simulink model "Ten_phase_nine_leg_relocated_L3_L7"  (R2025b)
settings: Solver=VariableStepAuto  StartTime=0.0  StopTime=0.05  FixedStep=1e-6  MaxStep=1e-6  RelTol=1e-4
values from neighbouring files (symbols this model uses):
  bias_current = 5    [parameters_for_AMB_topology.m]
  half_SW_Ts = SW_Ts*0.5    (= 2.5e-05)    [parameters_for_AMB_topology.m]
  K_i = 2*pi*f_c*R_value/U_dc    (= 47.1238898038)    [parameters_for_AMB_topology.m]
  K_p = 2*pi*f_c*L_value/U_dc    (= 0.0235619449019)    [parameters_for_AMB_topology.m]
  R_value = 1    [parameters_for_AMB_topology.m]
  SW_Ts = 1/(SW_frequency)    (= 5e-05)    [parameters_for_AMB_topology.m]
libraries: fl_lib x61, simulink x39, nesl_utility x29, eeGeneralControl x28, ee_lib x19
(part 3 of 4)

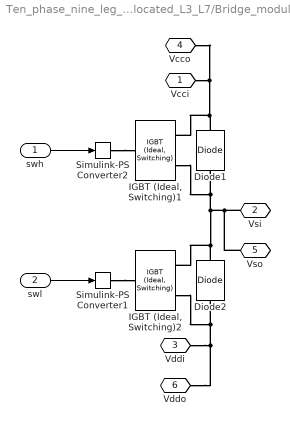
== system Ten_phase_nine_leg_relocated_L3_L7/Bridge_module6 ==
  swh : Inport
  swl : Inport  Port=2
  Diode1 : fl_lib/Electrical/Electrical Elements/Diode  Vf=0.6 V  Ron=0.3 Ohm  Goff=1e-8 1/Ohm  i_specify=off  i_priority=None  i=0 A  i_nominal_specify=off  i_nominal_value=1  i_nominal_unit=A  v_specify=off  v_priority=None  v=0 V  v_nominal_specify=off  v_nominal_value=1  v_nominal_unit=V
  Diode2 : fl_lib/Electrical/Electrical Elements/Diode  Vf=0.6 V  Ron=0.3 Ohm  Goff=1e-8 1/Ohm  i_specify=off  i_priority=None  i=0 A  i_nominal_specify=off  i_nominal_value=1  i_nominal_unit=A  v_specify=off  v_priority=None  v=0 V  v_nominal_specify=off  v_nominal_value=1  v_nominal_unit=V
  "IGBT (Ideal, Switching)1" : ee_lib/Semiconductors & Converters/IGBT (Ideal, Switching)  port_option=ee.enum.controlport.ps  Vf=0.8 V  Ron=0.001 Ohm  Goff=1e-5 1/Ohm  Vth=6 V  diode_param=ee.enum.semiconductors.protectionDiode.external  diode_Vf=0.8 V  diode_Ron=0.001 Ohm  diode_Goff=1e-5 1/Ohm  diode_C=50e-9 F  diode_iRM=-235 A  diode_iF=300 A  diode_idot=-50 A/us  diode_trr_param=ee.enum.converters.diodeReverseParam.trr_factor  diode_trr_factor=3  diode_trr=15 us  diode_Qrr=1500 s*uA  ice_specify=off  ice_priority=None  ice=0 A  ice_nominal_specify=off  ice_nominal_value=1  ice_nominal_unit=A  vce_specify=off  vce_priority=None  vce=0 V  vce_nominal_specify=off  vce_nominal_value=1  vce_nominal_unit=V  vge_specify=off  vge_priority=None  vge=0 V  vge_nominal_specify=off  vge_nominal_value=1  vge_nominal_unit=V  thermal_loss_option=ee.enum.converters.thermalLossOption.constantvalues  Von_data=[0, .1, .6, .8, 1, 1.3, 1.6, 2, 2.4; 0, .1, .7, 1, 1.2, 1.5, 1.9, 2.4, 2.8] V  Tj=[298.15, 398.15] K  Iout_data=[0, .1, 1, 5, 10, 20, 40, 70, 100] A  Eon_data=[0, .0024, .024, .12, .2, .48, 1.04, 2.16, 3.24; 0, .003, .03, .15, .25, .6, 1.3, 2.7, 4.05] * 1e-3 J  Eoff_data=[0, .0007, .0066, .033, .066, .17, .33, .83, 1.5; 0, .001, .01, .05, .1, .25, .5, 1.2, 2.2] * 1e-3 J  Eon_data_3D=[zeros(2, 9, 3)] J  Eoff_data_3D=[zeros(2, 9, 3)] J  Tj_loss=[298.15, 398.15] K  Iout_data_loss=[0, .1, 1, 5, 10, 20, 40, 70, 100] A  tabulateWithVce=false  Vce_loss=[0, 150, 300] V  Eon_scalar=22.86e-3 J  Eoff_scalar=17.14e-3 J  Voff=300 V  Iout_scalar=600 A  useCurrentFromPreviousCycle=false  useVoltageFromPreviousCycle=false  diodeModelType=ee.enum.converters.diodeModelType.pwl  diodeTableType=ee.enum.diode.tableType.IfMat  diode_ReverseIVType=ee.enum.diode.diodeReverseIV.constant  diode_IfMat=[.07, .12, .19, 1.75, 4.24, 7.32, 11.2; .16, .3, .72, 2.14, 4.02, 6.35, 9.12] A  diode_VfMat=[.9, 1.15, 1.25, 1.5, 1.75, 2.17, 2.6, 2.85; .58, .68, .75, 1.1, 1.38, 1.77, 2.27, 2.7] V  diode_TjVec=[25, 125] degC  diode_VfVec=[.5, .7, .9, 1.3, 1.7, 2.1, 2.5] V  diode_IfVec=[.1, .2, .5, 1, 2, 4, 7, 10] A  diode_IrMat=[1e-06, 2e-06, 5e-06, 1e-05, 2.5e-05, 5e-05, .0001; 2e-06, 5e-06, 1e-05, 4e-05, 8e-05, .0002, .0005] A  diode_VrMat=[10, 100, 200, 250, 300, 325, 350; 10, 70, 160, 220, 270, 300, 320] V  diode_VrVec=[10, 20, 40, 50, 70, 80, 100] V  diode_IrVec=[1e-06, 2e-06, 5e-06, 1e-05, 2e-05, 5e-05, .0001] A  diode_Vr=-600 V  diode_Ls=150 nH  diode_Erec=0.03 J  diode_rec_loss_model=ee.enum.diode.reverseRecoveryModel.fixed  diode_ErecVal=0 J  diode_scaleWithIandV=true  diode_ErecMat=zeros(2, 3) J  diode_TjrecVec=[298.15, 398.15] K  diode_IfrecVec=[.1, 1, 10] A  diode_IrecVal=10 A  diode_VrecVal=10 V  diode_tFilter=1 / 1000 / 100 s  separateThermalPortForDiode=false  thermal_network_parameterization=ee.enum.thermalNetworkTopology.external  Rth=[.08, .5] K/W  Rth_Cauer=[.08, .1, .5] K/W  Rth_Foster=[.08, .14, .22, .16] K/W  thermal_mass_parameterization=ee.enum.thermalNetwork.timeconstant  thermal_mass=[.01, .5] J/K  thermal_mass_Cauer=[.01, .1, .5] J/K  thermal_mass_Foster=[.001, .005, .05, .5] J/K  thermal_time_constant=[.001, .2] s  thermal_time_constant_Cauer=[.001, .1, .2] s  thermal_time_constant_Foster=[7e-05, .0007, .01, .08] s  thermal_mass_initial_temperatures=[25, 25] degC  thermal_mass_initial_temperatures_Cauer=[25, 25, 25] degC  junction_thermal_mass=0.01 J/K  Tvec_initial_Foster=[25, 25, 25, 25] degC  RthDiode=[.03, .2] K/W  RthCauerDiode=[.03, .1, .2] K/W  RthFosterDiode=[.03, .2] K/W  thermalMassDiode=[3, 25] J/K  thermalMassCauerDiode=[3, 10, 25] J/K  thermalMassFosterDiode=[33, 50] J/K  thermalTauDiode=[.1, 5] s  thermalTauCauerDiode=[.1, 1, 5] s  thermalTauFosterDiode=[1, 10] s  thermalMassInitTempDiode=[25, 25] degC  thermalMassInitTempCauerDiode=[25, 25, 25] degC  junctionthermalMassDiode=0.1 J/K  TVecInitialFosterDiode=[25, 25, 25, 25] degC  no_thermal_network=0  IGBT_junction_temperature_specify=off  IGBT_junction_temperature_priority=None  IGBT_junction_temperature=25 degC  IGBT_junction_temperature_nominal_specify=off  IGBT_junction_temperature_nominal_value=1  IGBT_junction_temperature_nominal_unit=degC  diode_junction_temperature_specify=off  diode_junction_temperature_priority=None  diode_junction_temperature=25 degC  diode_junction_temperature_nominal_specify=off  diode_junction_temperature_nominal_value=1  diode_junction_temperature_nominal_unit=degC  Qj_specify=off  Qj_priority=None  Qj=0 W  Qj_nominal_specify=off  Qj_nominal_value=1  Qj_nominal_unit=W  accumulatedSwitchingLosses_specify=off  accumulatedSwitchingLosses_priority=None  accumulatedSwitchingLosses=0 J
  "IGBT (Ideal, Switching)2" : ee_lib/Semiconductors & Converters/IGBT (Ideal, Switching)  port_option=ee.enum.controlport.ps  Vf=0.8 V  Ron=0.001 Ohm  Goff=1e-5 1/Ohm  Vth=6 V  diode_param=ee.enum.semiconductors.protectionDiode.external  diode_Vf=0.8 V  diode_Ron=0.001 Ohm  diode_Goff=1e-5 1/Ohm  diode_C=50e-9 F  diode_iRM=-235 A  diode_iF=300 A  diode_idot=-50 A/us  diode_trr_param=ee.enum.converters.diodeReverseParam.trr_factor  diode_trr_factor=3  diode_trr=15 us  diode_Qrr=1500 s*uA  ice_specify=off  ice_priority=None  ice=0 A  ice_nominal_specify=off  ice_nominal_value=1  ice_nominal_unit=A  vce_specify=off  vce_priority=None  vce=0 V  vce_nominal_specify=off  vce_nominal_value=1  vce_nominal_unit=V  vge_specify=off  vge_priority=None  vge=0 V  vge_nominal_specify=off  vge_nominal_value=1  vge_nominal_unit=V  thermal_loss_option=ee.enum.converters.thermalLossOption.constantvalues  Von_data=[0, .1, .6, .8, 1, 1.3, 1.6, 2, 2.4; 0, .1, .7, 1, 1.2, 1.5, 1.9, 2.4, 2.8] V  Tj=[298.15, 398.15] K  Iout_data=[0, .1, 1, 5, 10, 20, 40, 70, 100] A  Eon_data=[0, .0024, .024, .12, .2, .48, 1.04, 2.16, 3.24; 0, .003, .03, .15, .25, .6, 1.3, 2.7, 4.05] * 1e-3 J  Eoff_data=[0, .0007, .0066, .033, .066, .17, .33, .83, 1.5; 0, .001, .01, .05, .1, .25, .5, 1.2, 2.2] * 1e-3 J  Eon_data_3D=[zeros(2, 9, 3)] J  Eoff_data_3D=[zeros(2, 9, 3)] J  Tj_loss=[298.15, 398.15] K  Iout_data_loss=[0, .1, 1, 5, 10, 20, 40, 70, 100] A  tabulateWithVce=false  Vce_loss=[0, 150, 300] V  Eon_scalar=22.86e-3 J  Eoff_scalar=17.14e-3 J  Voff=300 V  Iout_scalar=600 A  useCurrentFromPreviousCycle=false  useVoltageFromPreviousCycle=false  diodeModelType=ee.enum.converters.diodeModelType.pwl  diodeTableType=ee.enum.diode.tableType.IfMat  diode_ReverseIVType=ee.enum.diode.diodeReverseIV.constant  diode_IfMat=[.07, .12, .19, 1.75, 4.24, 7.32, 11.2; .16, .3, .72, 2.14, 4.02, 6.35, 9.12] A  diode_VfMat=[.9, 1.15, 1.25, 1.5, 1.75, 2.17, 2.6, 2.85; .58, .68, .75, 1.1, 1.38, 1.77, 2.27, 2.7] V  diode_TjVec=[25, 125] degC  diode_VfVec=[.5, .7, .9, 1.3, 1.7, 2.1, 2.5] V  diode_IfVec=[.1, .2, .5, 1, 2, 4, 7, 10] A  diode_IrMat=[1e-06, 2e-06, 5e-06, 1e-05, 2.5e-05, 5e-05, .0001; 2e-06, 5e-06, 1e-05, 4e-05, 8e-05, .0002, .0005] A  diode_VrMat=[10, 100, 200, 250, 300, 325, 350; 10, 70, 160, 220, 270, 300, 320] V  diode_VrVec=[10, 20, 40, 50, 70, 80, 100] V  diode_IrVec=[1e-06, 2e-06, 5e-06, 1e-05, 2e-05, 5e-05, .0001] A  diode_Vr=-600 V  diode_Ls=150 nH  diode_Erec=0.03 J  diode_rec_loss_model=ee.enum.diode.reverseRecoveryModel.fixed  diode_ErecVal=0 J  diode_scaleWithIandV=true  diode_ErecMat=zeros(2, 3) J  diode_TjrecVec=[298.15, 398.15] K  diode_IfrecVec=[.1, 1, 10] A  diode_IrecVal=10 A  diode_VrecVal=10 V  diode_tFilter=1 / 1000 / 100 s  separateThermalPortForDiode=false  thermal_network_parameterization=ee.enum.thermalNetworkTopology.external  Rth=[.08, .5] K/W  Rth_Cauer=[.08, .1, .5] K/W  Rth_Foster=[.08, .14, .22, .16] K/W  thermal_mass_parameterization=ee.enum.thermalNetwork.timeconstant  thermal_mass=[.01, .5] J/K  thermal_mass_Cauer=[.01, .1, .5] J/K  thermal_mass_Foster=[.001, .005, .05, .5] J/K  thermal_time_constant=[.001, .2] s  thermal_time_constant_Cauer=[.001, .1, .2] s  thermal_time_constant_Foster=[7e-05, .0007, .01, .08] s  thermal_mass_initial_temperatures=[25, 25] degC  thermal_mass_initial_temperatures_Cauer=[25, 25, 25] degC  junction_thermal_mass=0.01 J/K  Tvec_initial_Foster=[25, 25, 25, 25] degC  RthDiode=[.03, .2] K/W  RthCauerDiode=[.03, .1, .2] K/W  RthFosterDiode=[.03, .2] K/W  thermalMassDiode=[3, 25] J/K  thermalMassCauerDiode=[3, 10, 25] J/K  thermalMassFosterDiode=[33, 50] J/K  thermalTauDiode=[.1, 5] s  thermalTauCauerDiode=[.1, 1, 5] s  thermalTauFosterDiode=[1, 10] s  thermalMassInitTempDiode=[25, 25] degC  thermalMassInitTempCauerDiode=[25, 25, 25] degC  junctionthermalMassDiode=0.1 J/K  TVecInitialFosterDiode=[25, 25, 25, 25] degC  no_thermal_network=0  IGBT_junction_temperature_specify=off  IGBT_junction_temperature_priority=None  IGBT_junction_temperature=25 degC  IGBT_junction_temperature_nominal_specify=off  IGBT_junction_temperature_nominal_value=1  IGBT_junction_temperature_nominal_unit=degC  diode_junction_temperature_specify=off  diode_junction_temperature_priority=None  diode_junction_temperature=25 degC  diode_junction_temperature_nominal_specify=off  diode_junction_temperature_nominal_value=1  diode_junction_temperature_nominal_unit=degC  Qj_specify=off  Qj_priority=None  Qj=0 W  Qj_nominal_specify=off  Qj_nominal_value=1  Qj_nominal_unit=W  accumulatedSwitchingLosses_specify=off  accumulatedSwitchingLosses_priority=None  accumulatedSwitchingLosses=0 J
  Simulink-PS Converter1 : nesl_utility/Simulink-PS Converter  PhysicalDomain=network_engine_domain  SubClassName=ps_input  LeftPortType=input  RightPortType=output  PseudoPeriodic=off  Frequencies=[]  NoiseDistribution=none  NoiseParameters=[]  Unit=1  AffineConversion=off  FilteringAndDerivatives=provide  SimscapeFilterOrder=1  InputFilterTimeConstant=0.001  UdotUserProvided=0
  Simulink-PS Converter2 : nesl_utility/Simulink-PS Converter  PhysicalDomain=network_engine_domain  SubClassName=ps_input  LeftPortType=input  RightPortType=output  PseudoPeriodic=off  Frequencies=[]  NoiseDistribution=none  NoiseParameters=[]  Unit=1  AffineConversion=off  FilteringAndDerivatives=provide  SimscapeFilterOrder=1  InputFilterTimeConstant=0.001  UdotUserProvided=0
  Vcci : PMIOPort  Side=Left
  Vsi : PMIOPort  Port=2  Side=Left
  Vddi : PMIOPort  Port=3  Side=Left
  Vcco : PMIOPort  Port=4  Side=Right
  Vso : PMIOPort  Port=5  Side=Right
  Vddo : PMIOPort  Port=6  Side=Right
  wires:
  swh/1 -> Simulink-PS Converter2/1
  swl/1 -> Simulink-PS Converter1/1
  connections:
  Diode1/RConn1 -- Vcco/RConn1 -- Vcci/RConn1 -- "IGBT (Ideal, Switching)1"/RConn1
  Simulink-PS Converter2/RConn1 -- "IGBT (Ideal, Switching)1"/LConn1
  "IGBT (Ideal, Switching)1"/RConn2 -- Vso/RConn1 -- Vsi/RConn1 -- "IGBT (Ideal, Switching)2"/RConn1 -- Diode2/RConn1 -- Diode1/LConn1
  "IGBT (Ideal, Switching)2"/RConn2 -- Vddo/RConn1 -- Vddi/RConn1 -- Diode2/LConn1
  Simulink-PS Converter1/RConn1 -- "IGBT (Ideal, Switching)2"/LConn1

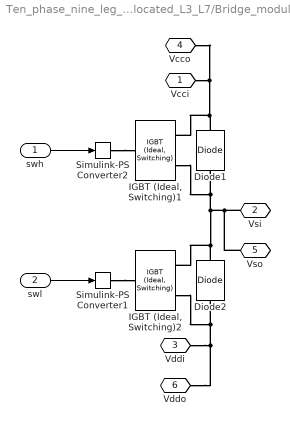
== system Ten_phase_nine_leg_relocated_L3_L7/Bridge_module7 ==
  swh : Inport
  swl : Inport  Port=2
  Diode1 : fl_lib/Electrical/Electrical Elements/Diode  Vf=0.6 V  Ron=0.3 Ohm  Goff=1e-8 1/Ohm  i_specify=off  i_priority=None  i=0 A  i_nominal_specify=off  i_nominal_value=1  i_nominal_unit=A  v_specify=off  v_priority=None  v=0 V  v_nominal_specify=off  v_nominal_value=1  v_nominal_unit=V
  Diode2 : fl_lib/Electrical/Electrical Elements/Diode  Vf=0.6 V  Ron=0.3 Ohm  Goff=1e-8 1/Ohm  i_specify=off  i_priority=None  i=0 A  i_nominal_specify=off  i_nominal_value=1  i_nominal_unit=A  v_specify=off  v_priority=None  v=0 V  v_nominal_specify=off  v_nominal_value=1  v_nominal_unit=V
  "IGBT (Ideal, Switching)1" : ee_lib/Semiconductors & Converters/IGBT (Ideal, Switching)  port_option=ee.enum.controlport.ps  Vf=0.8 V  Ron=0.001 Ohm  Goff=1e-5 1/Ohm  Vth=6 V  diode_param=ee.enum.semiconductors.protectionDiode.external  diode_Vf=0.8 V  diode_Ron=0.001 Ohm  diode_Goff=1e-5 1/Ohm  diode_C=50e-9 F  diode_iRM=-235 A  diode_iF=300 A  diode_idot=-50 A/us  diode_trr_param=ee.enum.converters.diodeReverseParam.trr_factor  diode_trr_factor=3  diode_trr=15 us  diode_Qrr=1500 s*uA  ice_specify=off  ice_priority=None  ice=0 A  ice_nominal_specify=off  ice_nominal_value=1  ice_nominal_unit=A  vce_specify=off  vce_priority=None  vce=0 V  vce_nominal_specify=off  vce_nominal_value=1  vce_nominal_unit=V  vge_specify=off  vge_priority=None  vge=0 V  vge_nominal_specify=off  vge_nominal_value=1  vge_nominal_unit=V  thermal_loss_option=ee.enum.converters.thermalLossOption.constantvalues  Von_data=[0, .1, .6, .8, 1, 1.3, 1.6, 2, 2.4; 0, .1, .7, 1, 1.2, 1.5, 1.9, 2.4, 2.8] V  Tj=[298.15, 398.15] K  Iout_data=[0, .1, 1, 5, 10, 20, 40, 70, 100] A  Eon_data=[0, .0024, .024, .12, .2, .48, 1.04, 2.16, 3.24; 0, .003, .03, .15, .25, .6, 1.3, 2.7, 4.05] * 1e-3 J  Eoff_data=[0, .0007, .0066, .033, .066, .17, .33, .83, 1.5; 0, .001, .01, .05, .1, .25, .5, 1.2, 2.2] * 1e-3 J  Eon_data_3D=[zeros(2, 9, 3)] J  Eoff_data_3D=[zeros(2, 9, 3)] J  Tj_loss=[298.15, 398.15] K  Iout_data_loss=[0, .1, 1, 5, 10, 20, 40, 70, 100] A  tabulateWithVce=false  Vce_loss=[0, 150, 300] V  Eon_scalar=22.86e-3 J  Eoff_scalar=17.14e-3 J  Voff=300 V  Iout_scalar=600 A  useCurrentFromPreviousCycle=false  useVoltageFromPreviousCycle=false  diodeModelType=ee.enum.converters.diodeModelType.pwl  diodeTableType=ee.enum.diode.tableType.IfMat  diode_ReverseIVType=ee.enum.diode.diodeReverseIV.constant  diode_IfMat=[.07, .12, .19, 1.75, 4.24, 7.32, 11.2; .16, .3, .72, 2.14, 4.02, 6.35, 9.12] A  diode_VfMat=[.9, 1.15, 1.25, 1.5, 1.75, 2.17, 2.6, 2.85; .58, .68, .75, 1.1, 1.38, 1.77, 2.27, 2.7] V  diode_TjVec=[25, 125] degC  diode_VfVec=[.5, .7, .9, 1.3, 1.7, 2.1, 2.5] V  diode_IfVec=[.1, .2, .5, 1, 2, 4, 7, 10] A  diode_IrMat=[1e-06, 2e-06, 5e-06, 1e-05, 2.5e-05, 5e-05, .0001; 2e-06, 5e-06, 1e-05, 4e-05, 8e-05, .0002, .0005] A  diode_VrMat=[10, 100, 200, 250, 300, 325, 350; 10, 70, 160, 220, 270, 300, 320] V  diode_VrVec=[10, 20, 40, 50, 70, 80, 100] V  diode_IrVec=[1e-06, 2e-06, 5e-06, 1e-05, 2e-05, 5e-05, .0001] A  diode_Vr=-600 V  diode_Ls=150 nH  diode_Erec=0.03 J  diode_rec_loss_model=ee.enum.diode.reverseRecoveryModel.fixed  diode_ErecVal=0 J  diode_scaleWithIandV=true  diode_ErecMat=zeros(2, 3) J  diode_TjrecVec=[298.15, 398.15] K  diode_IfrecVec=[.1, 1, 10] A  diode_IrecVal=10 A  diode_VrecVal=10 V  diode_tFilter=1 / 1000 / 100 s  separateThermalPortForDiode=false  thermal_network_parameterization=ee.enum.thermalNetworkTopology.external  Rth=[.08, .5] K/W  Rth_Cauer=[.08, .1, .5] K/W  Rth_Foster=[.08, .14, .22, .16] K/W  thermal_mass_parameterization=ee.enum.thermalNetwork.timeconstant  thermal_mass=[.01, .5] J/K  thermal_mass_Cauer=[.01, .1, .5] J/K  thermal_mass_Foster=[.001, .005, .05, .5] J/K  thermal_time_constant=[.001, .2] s  thermal_time_constant_Cauer=[.001, .1, .2] s  thermal_time_constant_Foster=[7e-05, .0007, .01, .08] s  thermal_mass_initial_temperatures=[25, 25] degC  thermal_mass_initial_temperatures_Cauer=[25, 25, 25] degC  junction_thermal_mass=0.01 J/K  Tvec_initial_Foster=[25, 25, 25, 25] degC  RthDiode=[.03, .2] K/W  RthCauerDiode=[.03, .1, .2] K/W  RthFosterDiode=[.03, .2] K/W  thermalMassDiode=[3, 25] J/K  thermalMassCauerDiode=[3, 10, 25] J/K  thermalMassFosterDiode=[33, 50] J/K  thermalTauDiode=[.1, 5] s  thermalTauCauerDiode=[.1, 1, 5] s  thermalTauFosterDiode=[1, 10] s  thermalMassInitTempDiode=[25, 25] degC  thermalMassInitTempCauerDiode=[25, 25, 25] degC  junctionthermalMassDiode=0.1 J/K  TVecInitialFosterDiode=[25, 25, 25, 25] degC  no_thermal_network=0  IGBT_junction_temperature_specify=off  IGBT_junction_temperature_priority=None  IGBT_junction_temperature=25 degC  IGBT_junction_temperature_nominal_specify=off  IGBT_junction_temperature_nominal_value=1  IGBT_junction_temperature_nominal_unit=degC  diode_junction_temperature_specify=off  diode_junction_temperature_priority=None  diode_junction_temperature=25 degC  diode_junction_temperature_nominal_specify=off  diode_junction_temperature_nominal_value=1  diode_junction_temperature_nominal_unit=degC  Qj_specify=off  Qj_priority=None  Qj=0 W  Qj_nominal_specify=off  Qj_nominal_value=1  Qj_nominal_unit=W  accumulatedSwitchingLosses_specify=off  accumulatedSwitchingLosses_priority=None  accumulatedSwitchingLosses=0 J
  "IGBT (Ideal, Switching)2" : ee_lib/Semiconductors & Converters/IGBT (Ideal, Switching)  port_option=ee.enum.controlport.ps  Vf=0.8 V  Ron=0.001 Ohm  Goff=1e-5 1/Ohm  Vth=6 V  diode_param=ee.enum.semiconductors.protectionDiode.external  diode_Vf=0.8 V  diode_Ron=0.001 Ohm  diode_Goff=1e-5 1/Ohm  diode_C=50e-9 F  diode_iRM=-235 A  diode_iF=300 A  diode_idot=-50 A/us  diode_trr_param=ee.enum.converters.diodeReverseParam.trr_factor  diode_trr_factor=3  diode_trr=15 us  diode_Qrr=1500 s*uA  ice_specify=off  ice_priority=None  ice=0 A  ice_nominal_specify=off  ice_nominal_value=1  ice_nominal_unit=A  vce_specify=off  vce_priority=None  vce=0 V  vce_nominal_specify=off  vce_nominal_value=1  vce_nominal_unit=V  vge_specify=off  vge_priority=None  vge=0 V  vge_nominal_specify=off  vge_nominal_value=1  vge_nominal_unit=V  thermal_loss_option=ee.enum.converters.thermalLossOption.constantvalues  Von_data=[0, .1, .6, .8, 1, 1.3, 1.6, 2, 2.4; 0, .1, .7, 1, 1.2, 1.5, 1.9, 2.4, 2.8] V  Tj=[298.15, 398.15] K  Iout_data=[0, .1, 1, 5, 10, 20, 40, 70, 100] A  Eon_data=[0, .0024, .024, .12, .2, .48, 1.04, 2.16, 3.24; 0, .003, .03, .15, .25, .6, 1.3, 2.7, 4.05] * 1e-3 J  Eoff_data=[0, .0007, .0066, .033, .066, .17, .33, .83, 1.5; 0, .001, .01, .05, .1, .25, .5, 1.2, 2.2] * 1e-3 J  Eon_data_3D=[zeros(2, 9, 3)] J  Eoff_data_3D=[zeros(2, 9, 3)] J  Tj_loss=[298.15, 398.15] K  Iout_data_loss=[0, .1, 1, 5, 10, 20, 40, 70, 100] A  tabulateWithVce=false  Vce_loss=[0, 150, 300] V  Eon_scalar=22.86e-3 J  Eoff_scalar=17.14e-3 J  Voff=300 V  Iout_scalar=600 A  useCurrentFromPreviousCycle=false  useVoltageFromPreviousCycle=false  diodeModelType=ee.enum.converters.diodeModelType.pwl  diodeTableType=ee.enum.diode.tableType.IfMat  diode_ReverseIVType=ee.enum.diode.diodeReverseIV.constant  diode_IfMat=[.07, .12, .19, 1.75, 4.24, 7.32, 11.2; .16, .3, .72, 2.14, 4.02, 6.35, 9.12] A  diode_VfMat=[.9, 1.15, 1.25, 1.5, 1.75, 2.17, 2.6, 2.85; .58, .68, .75, 1.1, 1.38, 1.77, 2.27, 2.7] V  diode_TjVec=[25, 125] degC  diode_VfVec=[.5, .7, .9, 1.3, 1.7, 2.1, 2.5] V  diode_IfVec=[.1, .2, .5, 1, 2, 4, 7, 10] A  diode_IrMat=[1e-06, 2e-06, 5e-06, 1e-05, 2.5e-05, 5e-05, .0001; 2e-06, 5e-06, 1e-05, 4e-05, 8e-05, .0002, .0005] A  diode_VrMat=[10, 100, 200, 250, 300, 325, 350; 10, 70, 160, 220, 270, 300, 320] V  diode_VrVec=[10, 20, 40, 50, 70, 80, 100] V  diode_IrVec=[1e-06, 2e-06, 5e-06, 1e-05, 2e-05, 5e-05, .0001] A  diode_Vr=-600 V  diode_Ls=150 nH  diode_Erec=0.03 J  diode_rec_loss_model=ee.enum.diode.reverseRecoveryModel.fixed  diode_ErecVal=0 J  diode_scaleWithIandV=true  diode_ErecMat=zeros(2, 3) J  diode_TjrecVec=[298.15, 398.15] K  diode_IfrecVec=[.1, 1, 10] A  diode_IrecVal=10 A  diode_VrecVal=10 V  diode_tFilter=1 / 1000 / 100 s  separateThermalPortForDiode=false  thermal_network_parameterization=ee.enum.thermalNetworkTopology.external  Rth=[.08, .5] K/W  Rth_Cauer=[.08, .1, .5] K/W  Rth_Foster=[.08, .14, .22, .16] K/W  thermal_mass_parameterization=ee.enum.thermalNetwork.timeconstant  thermal_mass=[.01, .5] J/K  thermal_mass_Cauer=[.01, .1, .5] J/K  thermal_mass_Foster=[.001, .005, .05, .5] J/K  thermal_time_constant=[.001, .2] s  thermal_time_constant_Cauer=[.001, .1, .2] s  thermal_time_constant_Foster=[7e-05, .0007, .01, .08] s  thermal_mass_initial_temperatures=[25, 25] degC  thermal_mass_initial_temperatures_Cauer=[25, 25, 25] degC  junction_thermal_mass=0.01 J/K  Tvec_initial_Foster=[25, 25, 25, 25] degC  RthDiode=[.03, .2] K/W  RthCauerDiode=[.03, .1, .2] K/W  RthFosterDiode=[.03, .2] K/W  thermalMassDiode=[3, 25] J/K  thermalMassCauerDiode=[3, 10, 25] J/K  thermalMassFosterDiode=[33, 50] J/K  thermalTauDiode=[.1, 5] s  thermalTauCauerDiode=[.1, 1, 5] s  thermalTauFosterDiode=[1, 10] s  thermalMassInitTempDiode=[25, 25] degC  thermalMassInitTempCauerDiode=[25, 25, 25] degC  junctionthermalMassDiode=0.1 J/K  TVecInitialFosterDiode=[25, 25, 25, 25] degC  no_thermal_network=0  IGBT_junction_temperature_specify=off  IGBT_junction_temperature_priority=None  IGBT_junction_temperature=25 degC  IGBT_junction_temperature_nominal_specify=off  IGBT_junction_temperature_nominal_value=1  IGBT_junction_temperature_nominal_unit=degC  diode_junction_temperature_specify=off  diode_junction_temperature_priority=None  diode_junction_temperature=25 degC  diode_junction_temperature_nominal_specify=off  diode_junction_temperature_nominal_value=1  diode_junction_temperature_nominal_unit=degC  Qj_specify=off  Qj_priority=None  Qj=0 W  Qj_nominal_specify=off  Qj_nominal_value=1  Qj_nominal_unit=W  accumulatedSwitchingLosses_specify=off  accumulatedSwitchingLosses_priority=None  accumulatedSwitchingLosses=0 J
  Simulink-PS Converter1 : nesl_utility/Simulink-PS Converter  PhysicalDomain=network_engine_domain  SubClassName=ps_input  LeftPortType=input  RightPortType=output  PseudoPeriodic=off  Frequencies=[]  NoiseDistribution=none  NoiseParameters=[]  Unit=1  AffineConversion=off  FilteringAndDerivatives=provide  SimscapeFilterOrder=1  InputFilterTimeConstant=0.001  UdotUserProvided=0
  Simulink-PS Converter2 : nesl_utility/Simulink-PS Converter  PhysicalDomain=network_engine_domain  SubClassName=ps_input  LeftPortType=input  RightPortType=output  PseudoPeriodic=off  Frequencies=[]  NoiseDistribution=none  NoiseParameters=[]  Unit=1  AffineConversion=off  FilteringAndDerivatives=provide  SimscapeFilterOrder=1  InputFilterTimeConstant=0.001  UdotUserProvided=0
  Vcci : PMIOPort  Side=Left
  Vsi : PMIOPort  Port=2  Side=Left
  Vddi : PMIOPort  Port=3  Side=Left
  Vcco : PMIOPort  Port=4  Side=Right
  Vso : PMIOPort  Port=5  Side=Right
  Vddo : PMIOPort  Port=6  Side=Right
  wires:
  swh/1 -> Simulink-PS Converter2/1
  swl/1 -> Simulink-PS Converter1/1
  connections:
  Diode1/RConn1 -- Vcco/RConn1 -- Vcci/RConn1 -- "IGBT (Ideal, Switching)1"/RConn1
  Simulink-PS Converter2/RConn1 -- "IGBT (Ideal, Switching)1"/LConn1
  "IGBT (Ideal, Switching)1"/RConn2 -- Vso/RConn1 -- Vsi/RConn1 -- "IGBT (Ideal, Switching)2"/RConn1 -- Diode2/RConn1 -- Diode1/LConn1
  "IGBT (Ideal, Switching)2"/RConn2 -- Vddo/RConn1 -- Vddi/RConn1 -- Diode2/LConn1
  Simulink-PS Converter1/RConn1 -- "IGBT (Ideal, Switching)2"/LConn1

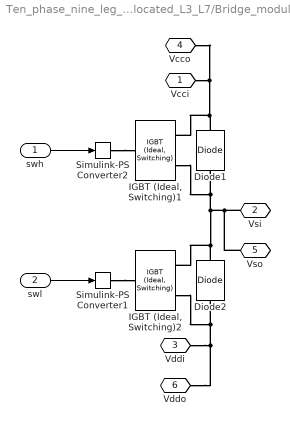
== system Ten_phase_nine_leg_relocated_L3_L7/Bridge_module8 ==
  swh : Inport
  swl : Inport  Port=2
  Diode1 : fl_lib/Electrical/Electrical Elements/Diode  Vf=0.6 V  Ron=0.3 Ohm  Goff=1e-8 1/Ohm  i_specify=off  i_priority=None  i=0 A  i_nominal_specify=off  i_nominal_value=1  i_nominal_unit=A  v_specify=off  v_priority=None  v=0 V  v_nominal_specify=off  v_nominal_value=1  v_nominal_unit=V
  Diode2 : fl_lib/Electrical/Electrical Elements/Diode  Vf=0.6 V  Ron=0.3 Ohm  Goff=1e-8 1/Ohm  i_specify=off  i_priority=None  i=0 A  i_nominal_specify=off  i_nominal_value=1  i_nominal_unit=A  v_specify=off  v_priority=None  v=0 V  v_nominal_specify=off  v_nominal_value=1  v_nominal_unit=V
  "IGBT (Ideal, Switching)1" : ee_lib/Semiconductors & Converters/IGBT (Ideal, Switching)  port_option=ee.enum.controlport.ps  Vf=0.8 V  Ron=0.001 Ohm  Goff=1e-5 1/Ohm  Vth=6 V  diode_param=ee.enum.semiconductors.protectionDiode.external  diode_Vf=0.8 V  diode_Ron=0.001 Ohm  diode_Goff=1e-5 1/Ohm  diode_C=50e-9 F  diode_iRM=-235 A  diode_iF=300 A  diode_idot=-50 A/us  diode_trr_param=ee.enum.converters.diodeReverseParam.trr_factor  diode_trr_factor=3  diode_trr=15 us  diode_Qrr=1500 s*uA  ice_specify=off  ice_priority=None  ice=0 A  ice_nominal_specify=off  ice_nominal_value=1  ice_nominal_unit=A  vce_specify=off  vce_priority=None  vce=0 V  vce_nominal_specify=off  vce_nominal_value=1  vce_nominal_unit=V  vge_specify=off  vge_priority=None  vge=0 V  vge_nominal_specify=off  vge_nominal_value=1  vge_nominal_unit=V  thermal_loss_option=ee.enum.converters.thermalLossOption.constantvalues  Von_data=[0, .1, .6, .8, 1, 1.3, 1.6, 2, 2.4; 0, .1, .7, 1, 1.2, 1.5, 1.9, 2.4, 2.8] V  Tj=[298.15, 398.15] K  Iout_data=[0, .1, 1, 5, 10, 20, 40, 70, 100] A  Eon_data=[0, .0024, .024, .12, .2, .48, 1.04, 2.16, 3.24; 0, .003, .03, .15, .25, .6, 1.3, 2.7, 4.05] * 1e-3 J  Eoff_data=[0, .0007, .0066, .033, .066, .17, .33, .83, 1.5; 0, .001, .01, .05, .1, .25, .5, 1.2, 2.2] * 1e-3 J  Eon_data_3D=[zeros(2, 9, 3)] J  Eoff_data_3D=[zeros(2, 9, 3)] J  Tj_loss=[298.15, 398.15] K  Iout_data_loss=[0, .1, 1, 5, 10, 20, 40, 70, 100] A  tabulateWithVce=false  Vce_loss=[0, 150, 300] V  Eon_scalar=22.86e-3 J  Eoff_scalar=17.14e-3 J  Voff=300 V  Iout_scalar=600 A  useCurrentFromPreviousCycle=false  useVoltageFromPreviousCycle=false  diodeModelType=ee.enum.converters.diodeModelType.pwl  diodeTableType=ee.enum.diode.tableType.IfMat  diode_ReverseIVType=ee.enum.diode.diodeReverseIV.constant  diode_IfMat=[.07, .12, .19, 1.75, 4.24, 7.32, 11.2; .16, .3, .72, 2.14, 4.02, 6.35, 9.12] A  diode_VfMat=[.9, 1.15, 1.25, 1.5, 1.75, 2.17, 2.6, 2.85; .58, .68, .75, 1.1, 1.38, 1.77, 2.27, 2.7] V  diode_TjVec=[25, 125] degC  diode_VfVec=[.5, .7, .9, 1.3, 1.7, 2.1, 2.5] V  diode_IfVec=[.1, .2, .5, 1, 2, 4, 7, 10] A  diode_IrMat=[1e-06, 2e-06, 5e-06, 1e-05, 2.5e-05, 5e-05, .0001; 2e-06, 5e-06, 1e-05, 4e-05, 8e-05, .0002, .0005] A  diode_VrMat=[10, 100, 200, 250, 300, 325, 350; 10, 70, 160, 220, 270, 300, 320] V  diode_VrVec=[10, 20, 40, 50, 70, 80, 100] V  diode_IrVec=[1e-06, 2e-06, 5e-06, 1e-05, 2e-05, 5e-05, .0001] A  diode_Vr=-600 V  diode_Ls=150 nH  diode_Erec=0.03 J  diode_rec_loss_model=ee.enum.diode.reverseRecoveryModel.fixed  diode_ErecVal=0 J  diode_scaleWithIandV=true  diode_ErecMat=zeros(2, 3) J  diode_TjrecVec=[298.15, 398.15] K  diode_IfrecVec=[.1, 1, 10] A  diode_IrecVal=10 A  diode_VrecVal=10 V  diode_tFilter=1 / 1000 / 100 s  separateThermalPortForDiode=false  thermal_network_parameterization=ee.enum.thermalNetworkTopology.external  Rth=[.08, .5] K/W  Rth_Cauer=[.08, .1, .5] K/W  Rth_Foster=[.08, .14, .22, .16] K/W  thermal_mass_parameterization=ee.enum.thermalNetwork.timeconstant  thermal_mass=[.01, .5] J/K  thermal_mass_Cauer=[.01, .1, .5] J/K  thermal_mass_Foster=[.001, .005, .05, .5] J/K  thermal_time_constant=[.001, .2] s  thermal_time_constant_Cauer=[.001, .1, .2] s  thermal_time_constant_Foster=[7e-05, .0007, .01, .08] s  thermal_mass_initial_temperatures=[25, 25] degC  thermal_mass_initial_temperatures_Cauer=[25, 25, 25] degC  junction_thermal_mass=0.01 J/K  Tvec_initial_Foster=[25, 25, 25, 25] degC  RthDiode=[.03, .2] K/W  RthCauerDiode=[.03, .1, .2] K/W  RthFosterDiode=[.03, .2] K/W  thermalMassDiode=[3, 25] J/K  thermalMassCauerDiode=[3, 10, 25] J/K  thermalMassFosterDiode=[33, 50] J/K  thermalTauDiode=[.1, 5] s  thermalTauCauerDiode=[.1, 1, 5] s  thermalTauFosterDiode=[1, 10] s  thermalMassInitTempDiode=[25, 25] degC  thermalMassInitTempCauerDiode=[25, 25, 25] degC  junctionthermalMassDiode=0.1 J/K  TVecInitialFosterDiode=[25, 25, 25, 25] degC  no_thermal_network=0  IGBT_junction_temperature_specify=off  IGBT_junction_temperature_priority=None  IGBT_junction_temperature=25 degC  IGBT_junction_temperature_nominal_specify=off  IGBT_junction_temperature_nominal_value=1  IGBT_junction_temperature_nominal_unit=degC  diode_junction_temperature_specify=off  diode_junction_temperature_priority=None  diode_junction_temperature=25 degC  diode_junction_temperature_nominal_specify=off  diode_junction_temperature_nominal_value=1  diode_junction_temperature_nominal_unit=degC  Qj_specify=off  Qj_priority=None  Qj=0 W  Qj_nominal_specify=off  Qj_nominal_value=1  Qj_nominal_unit=W  accumulatedSwitchingLosses_specify=off  accumulatedSwitchingLosses_priority=None  accumulatedSwitchingLosses=0 J
  "IGBT (Ideal, Switching)2" : ee_lib/Semiconductors & Converters/IGBT (Ideal, Switching)  port_option=ee.enum.controlport.ps  Vf=0.8 V  Ron=0.001 Ohm  Goff=1e-5 1/Ohm  Vth=6 V  diode_param=ee.enum.semiconductors.protectionDiode.external  diode_Vf=0.8 V  diode_Ron=0.001 Ohm  diode_Goff=1e-5 1/Ohm  diode_C=50e-9 F  diode_iRM=-235 A  diode_iF=300 A  diode_idot=-50 A/us  diode_trr_param=ee.enum.converters.diodeReverseParam.trr_factor  diode_trr_factor=3  diode_trr=15 us  diode_Qrr=1500 s*uA  ice_specify=off  ice_priority=None  ice=0 A  ice_nominal_specify=off  ice_nominal_value=1  ice_nominal_unit=A  vce_specify=off  vce_priority=None  vce=0 V  vce_nominal_specify=off  vce_nominal_value=1  vce_nominal_unit=V  vge_specify=off  vge_priority=None  vge=0 V  vge_nominal_specify=off  vge_nominal_value=1  vge_nominal_unit=V  thermal_loss_option=ee.enum.converters.thermalLossOption.constantvalues  Von_data=[0, .1, .6, .8, 1, 1.3, 1.6, 2, 2.4; 0, .1, .7, 1, 1.2, 1.5, 1.9, 2.4, 2.8] V  Tj=[298.15, 398.15] K  Iout_data=[0, .1, 1, 5, 10, 20, 40, 70, 100] A  Eon_data=[0, .0024, .024, .12, .2, .48, 1.04, 2.16, 3.24; 0, .003, .03, .15, .25, .6, 1.3, 2.7, 4.05] * 1e-3 J  Eoff_data=[0, .0007, .0066, .033, .066, .17, .33, .83, 1.5; 0, .001, .01, .05, .1, .25, .5, 1.2, 2.2] * 1e-3 J  Eon_data_3D=[zeros(2, 9, 3)] J  Eoff_data_3D=[zeros(2, 9, 3)] J  Tj_loss=[298.15, 398.15] K  Iout_data_loss=[0, .1, 1, 5, 10, 20, 40, 70, 100] A  tabulateWithVce=false  Vce_loss=[0, 150, 300] V  Eon_scalar=22.86e-3 J  Eoff_scalar=17.14e-3 J  Voff=300 V  Iout_scalar=600 A  useCurrentFromPreviousCycle=false  useVoltageFromPreviousCycle=false  diodeModelType=ee.enum.converters.diodeModelType.pwl  diodeTableType=ee.enum.diode.tableType.IfMat  diode_ReverseIVType=ee.enum.diode.diodeReverseIV.constant  diode_IfMat=[.07, .12, .19, 1.75, 4.24, 7.32, 11.2; .16, .3, .72, 2.14, 4.02, 6.35, 9.12] A  diode_VfMat=[.9, 1.15, 1.25, 1.5, 1.75, 2.17, 2.6, 2.85; .58, .68, .75, 1.1, 1.38, 1.77, 2.27, 2.7] V  diode_TjVec=[25, 125] degC  diode_VfVec=[.5, .7, .9, 1.3, 1.7, 2.1, 2.5] V  diode_IfVec=[.1, .2, .5, 1, 2, 4, 7, 10] A  diode_IrMat=[1e-06, 2e-06, 5e-06, 1e-05, 2.5e-05, 5e-05, .0001; 2e-06, 5e-06, 1e-05, 4e-05, 8e-05, .0002, .0005] A  diode_VrMat=[10, 100, 200, 250, 300, 325, 350; 10, 70, 160, 220, 270, 300, 320] V  diode_VrVec=[10, 20, 40, 50, 70, 80, 100] V  diode_IrVec=[1e-06, 2e-06, 5e-06, 1e-05, 2e-05, 5e-05, .0001] A  diode_Vr=-600 V  diode_Ls=150 nH  diode_Erec=0.03 J  diode_rec_loss_model=ee.enum.diode.reverseRecoveryModel.fixed  diode_ErecVal=0 J  diode_scaleWithIandV=true  diode_ErecMat=zeros(2, 3) J  diode_TjrecVec=[298.15, 398.15] K  diode_IfrecVec=[.1, 1, 10] A  diode_IrecVal=10 A  diode_VrecVal=10 V  diode_tFilter=1 / 1000 / 100 s  separateThermalPortForDiode=false  thermal_network_parameterization=ee.enum.thermalNetworkTopology.external  Rth=[.08, .5] K/W  Rth_Cauer=[.08, .1, .5] K/W  Rth_Foster=[.08, .14, .22, .16] K/W  thermal_mass_parameterization=ee.enum.thermalNetwork.timeconstant  thermal_mass=[.01, .5] J/K  thermal_mass_Cauer=[.01, .1, .5] J/K  thermal_mass_Foster=[.001, .005, .05, .5] J/K  thermal_time_constant=[.001, .2] s  thermal_time_constant_Cauer=[.001, .1, .2] s  thermal_time_constant_Foster=[7e-05, .0007, .01, .08] s  thermal_mass_initial_temperatures=[25, 25] degC  thermal_mass_initial_temperatures_Cauer=[25, 25, 25] degC  junction_thermal_mass=0.01 J/K  Tvec_initial_Foster=[25, 25, 25, 25] degC  RthDiode=[.03, .2] K/W  RthCauerDiode=[.03, .1, .2] K/W  RthFosterDiode=[.03, .2] K/W  thermalMassDiode=[3, 25] J/K  thermalMassCauerDiode=[3, 10, 25] J/K  thermalMassFosterDiode=[33, 50] J/K  thermalTauDiode=[.1, 5] s  thermalTauCauerDiode=[.1, 1, 5] s  thermalTauFosterDiode=[1, 10] s  thermalMassInitTempDiode=[25, 25] degC  thermalMassInitTempCauerDiode=[25, 25, 25] degC  junctionthermalMassDiode=0.1 J/K  TVecInitialFosterDiode=[25, 25, 25, 25] degC  no_thermal_network=0  IGBT_junction_temperature_specify=off  IGBT_junction_temperature_priority=None  IGBT_junction_temperature=25 degC  IGBT_junction_temperature_nominal_specify=off  IGBT_junction_temperature_nominal_value=1  IGBT_junction_temperature_nominal_unit=degC  diode_junction_temperature_specify=off  diode_junction_temperature_priority=None  diode_junction_temperature=25 degC  diode_junction_temperature_nominal_specify=off  diode_junction_temperature_nominal_value=1  diode_junction_temperature_nominal_unit=degC  Qj_specify=off  Qj_priority=None  Qj=0 W  Qj_nominal_specify=off  Qj_nominal_value=1  Qj_nominal_unit=W  accumulatedSwitchingLosses_specify=off  accumulatedSwitchingLosses_priority=None  accumulatedSwitchingLosses=0 J
  Simulink-PS Converter1 : nesl_utility/Simulink-PS Converter  PhysicalDomain=network_engine_domain  SubClassName=ps_input  LeftPortType=input  RightPortType=output  PseudoPeriodic=off  Frequencies=[]  NoiseDistribution=none  NoiseParameters=[]  Unit=1  AffineConversion=off  FilteringAndDerivatives=provide  SimscapeFilterOrder=1  InputFilterTimeConstant=0.001  UdotUserProvided=0
  Simulink-PS Converter2 : nesl_utility/Simulink-PS Converter  PhysicalDomain=network_engine_domain  SubClassName=ps_input  LeftPortType=input  RightPortType=output  PseudoPeriodic=off  Frequencies=[]  NoiseDistribution=none  NoiseParameters=[]  Unit=1  AffineConversion=off  FilteringAndDerivatives=provide  SimscapeFilterOrder=1  InputFilterTimeConstant=0.001  UdotUserProvided=0
  Vcci : PMIOPort  Side=Left
  Vsi : PMIOPort  Port=2  Side=Left
  Vddi : PMIOPort  Port=3  Side=Left
  Vcco : PMIOPort  Port=4  Side=Right
  Vso : PMIOPort  Port=5  Side=Right
  Vddo : PMIOPort  Port=6  Side=Right
  wires:
  swh/1 -> Simulink-PS Converter2/1
  swl/1 -> Simulink-PS Converter1/1
  connections:
  Diode1/RConn1 -- Vcco/RConn1 -- Vcci/RConn1 -- "IGBT (Ideal, Switching)1"/RConn1
  Simulink-PS Converter2/RConn1 -- "IGBT (Ideal, Switching)1"/LConn1
  "IGBT (Ideal, Switching)1"/RConn2 -- Vso/RConn1 -- Vsi/RConn1 -- "IGBT (Ideal, Switching)2"/RConn1 -- Diode2/RConn1 -- Diode1/LConn1
  "IGBT (Ideal, Switching)2"/RConn2 -- Vddo/RConn1 -- Vddi/RConn1 -- Diode2/LConn1
  Simulink-PS Converter1/RConn1 -- "IGBT (Ideal, Switching)2"/LConn1

== system Ten_phase_nine_leg_relocated_L3_L7/PI_ctrl ==
  ref : Inport
  fbk : Inport  Port=2
  Add2 : Sum  Inputs=+-
  Add3 : Sum
  Gain4 : Gain  Gain=K_p
  Ictrl_anti_windup : Subsystem
  Memory : Memory
  Rate Transition : RateTransition  OutPortSampleTime=SW_Ts
  Saturation : Saturate  UpperLimit=1  LowerLimit=-1
  Second-Order Filter : eeGeneralControl/Second-Order Filter  FilterType=Low-pass  fn=6000  Zeta=0.707  Ts=0  A0=0  Ph0=0  f0=0  b0=0
      settings: LibrarySourceBlock=ee_sl_lib/General Control/Second-Order Filter
  U_cmd : Outport
  wires:
  Gain4/1 -> Add3/1
  Memory/1 -> Second-Order Filter/1
  Second-Order Filter/1 -> Add2/2
  Saturation/1 -> U_cmd/1
  Add2/1 -> Ictrl_anti_windup/1(err), Gain4/1
  Add3/1 -> Saturation/1
  ref/1 -> Add2/1
  fbk/1 -> Rate Transition/1
  Rate Transition/1 -> Memory/1
  Ictrl_anti_windup/1(Int_out) -> Add3/2

== system Ten_phase_nine_leg_relocated_L3_L7/PI_ctrl1 ==
  ref : Inport
  fbk : Inport  Port=2
  Add2 : Sum  Inputs=+-
  Add3 : Sum
  Gain4 : Gain  Gain=K_p
  Ictrl_anti_windup : Subsystem
  Memory : Memory
  Rate Transition : RateTransition  OutPortSampleTime=SW_Ts
  Saturation : Saturate  UpperLimit=1  LowerLimit=-1
  Second-Order Filter : eeGeneralControl/Second-Order Filter  FilterType=Low-pass  fn=6000  Zeta=0.707  Ts=0  A0=0  Ph0=0  f0=0  b0=0
      settings: LibrarySourceBlock=ee_sl_lib/General Control/Second-Order Filter
  U_cmd : Outport
  wires:
  Gain4/1 -> Add3/1
  Memory/1 -> Second-Order Filter/1
  Second-Order Filter/1 -> Add2/2
  Saturation/1 -> U_cmd/1
  Add2/1 -> Ictrl_anti_windup/1(err), Gain4/1
  Add3/1 -> Saturation/1
  ref/1 -> Add2/1
  fbk/1 -> Rate Transition/1
  Rate Transition/1 -> Memory/1
  Ictrl_anti_windup/1(Int_out) -> Add3/2

== system Ten_phase_nine_leg_relocated_L3_L7/PI_ctrl2 ==
  ref : Inport
  fbk : Inport  Port=2
  Add2 : Sum  Inputs=+-
  Add3 : Sum
  Gain4 : Gain  Gain=K_p
  Ictrl_anti_windup : Subsystem
  Memory : Memory
  Rate Transition : RateTransition  OutPortSampleTime=SW_Ts
  Saturation : Saturate  UpperLimit=1  LowerLimit=-1
  Second-Order Filter : eeGeneralControl/Second-Order Filter  FilterType=Low-pass  fn=6000  Zeta=0.707  Ts=0  A0=0  Ph0=0  f0=0  b0=0
      settings: LibrarySourceBlock=ee_sl_lib/General Control/Second-Order Filter
  U_cmd : Outport
  wires:
  Gain4/1 -> Add3/1
  Memory/1 -> Second-Order Filter/1
  Second-Order Filter/1 -> Add2/2
  Saturation/1 -> U_cmd/1
  Add2/1 -> Ictrl_anti_windup/1(err), Gain4/1
  Add3/1 -> Saturation/1
  ref/1 -> Add2/1
  fbk/1 -> Rate Transition/1
  Rate Transition/1 -> Memory/1
  Ictrl_anti_windup/1(Int_out) -> Add3/2

== system Ten_phase_nine_leg_relocated_L3_L7/PI_ctrl3 ==
  ref : Inport
  fbk : Inport  Port=2
  Add2 : Sum  Inputs=+-
  Add3 : Sum
  Gain4 : Gain  Gain=K_p
  Ictrl_anti_windup : Subsystem
  Memory : Memory
  Rate Transition : RateTransition  OutPortSampleTime=SW_Ts
  Saturation : Saturate  UpperLimit=1  LowerLimit=-1
  Second-Order Filter : eeGeneralControl/Second-Order Filter  FilterType=Low-pass  fn=6000  Zeta=0.707  Ts=0  A0=0  Ph0=0  f0=0  b0=0
      settings: LibrarySourceBlock=ee_sl_lib/General Control/Second-Order Filter
  U_cmd : Outport
  wires:
  Gain4/1 -> Add3/1
  Memory/1 -> Second-Order Filter/1
  Second-Order Filter/1 -> Add2/2
  Saturation/1 -> U_cmd/1
  Add2/1 -> Ictrl_anti_windup/1(err), Gain4/1
  Add3/1 -> Saturation/1
  ref/1 -> Add2/1
  fbk/1 -> Rate Transition/1
  Rate Transition/1 -> Memory/1
  Ictrl_anti_windup/1(Int_out) -> Add3/2

== system Ten_phase_nine_leg_relocated_L3_L7/PI_ctrl4 ==
  ref : Inport
  fbk : Inport  Port=2
  Add2 : Sum  Inputs=+-
  Add3 : Sum
  Gain4 : Gain  Gain=K_p
  Ictrl_anti_windup : Subsystem
  Memory : Memory
  Rate Transition : RateTransition  OutPortSampleTime=SW_Ts
  Saturation : Saturate  UpperLimit=1  LowerLimit=-1
  Second-Order Filter : eeGeneralControl/Second-Order Filter  FilterType=Low-pass  fn=6000  Zeta=0.707  Ts=0  A0=0  Ph0=0  f0=0  b0=0
      settings: LibrarySourceBlock=ee_sl_lib/General Control/Second-Order Filter
  U_cmd : Outport
  wires:
  Gain4/1 -> Add3/1
  Memory/1 -> Second-Order Filter/1
  Second-Order Filter/1 -> Add2/2
  Saturation/1 -> U_cmd/1
  Add2/1 -> Ictrl_anti_windup/1(err), Gain4/1
  Add3/1 -> Saturation/1
  ref/1 -> Add2/1
  fbk/1 -> Rate Transition/1
  Rate Transition/1 -> Memory/1
  Ictrl_anti_windup/1(Int_out) -> Add3/2

== system Ten_phase_nine_leg_relocated_L3_L7/PI_ctrl5 ==
  ref : Inport
  fbk : Inport  Port=2
  Add2 : Sum  Inputs=+-
  Add3 : Sum
  Gain4 : Gain  Gain=K_p
  Ictrl_anti_windup : Subsystem
  Memory : Memory
  Rate Transition : RateTransition  OutPortSampleTime=SW_Ts
  Saturation : Saturate  UpperLimit=1  LowerLimit=-1
  Second-Order Filter : eeGeneralControl/Second-Order Filter  FilterType=Low-pass  fn=6000  Zeta=0.707  Ts=0  A0=0  Ph0=0  f0=0  b0=0
      settings: LibrarySourceBlock=ee_sl_lib/General Control/Second-Order Filter
  U_cmd : Outport
  wires:
  Gain4/1 -> Add3/1
  Memory/1 -> Second-Order Filter/1
  Second-Order Filter/1 -> Add2/2
  Saturation/1 -> U_cmd/1
  Add2/1 -> Ictrl_anti_windup/1(err), Gain4/1
  Add3/1 -> Saturation/1
  ref/1 -> Add2/1
  fbk/1 -> Rate Transition/1
  Rate Transition/1 -> Memory/1
  Ictrl_anti_windup/1(Int_out) -> Add3/2

== system Ten_phase_nine_leg_relocated_L3_L7/PI_ctrl6 ==
  ref : Inport
  fbk : Inport  Port=2
  Add2 : Sum  Inputs=+-
  Add3 : Sum
  Gain4 : Gain  Gain=K_p
  Ictrl_anti_windup : Subsystem
  Memory : Memory
  Rate Transition : RateTransition  OutPortSampleTime=SW_Ts
  Saturation : Saturate  UpperLimit=1  LowerLimit=-1
  Second-Order Filter : eeGeneralControl/Second-Order Filter  FilterType=Low-pass  fn=6000  Zeta=0.707  Ts=0  A0=0  Ph0=0  f0=0  b0=0
      settings: LibrarySourceBlock=ee_sl_lib/General Control/Second-Order Filter
  U_cmd : Outport
  wires:
  Gain4/1 -> Add3/1
  Memory/1 -> Second-Order Filter/1
  Second-Order Filter/1 -> Add2/2
  Saturation/1 -> U_cmd/1
  Add2/1 -> Ictrl_anti_windup/1(err), Gain4/1
  Add3/1 -> Saturation/1
  ref/1 -> Add2/1
  fbk/1 -> Rate Transition/1
  Rate Transition/1 -> Memory/1
  Ictrl_anti_windup/1(Int_out) -> Add3/2

== system Ten_phase_nine_leg_relocated_L3_L7/PI_ctrl7 ==
  ref : Inport
  fbk : Inport  Port=2
  Add2 : Sum  Inputs=+-
  Add3 : Sum
  Gain4 : Gain  Gain=K_p
  Ictrl_anti_windup : Subsystem
  Memory : Memory
  Rate Transition : RateTransition  OutPortSampleTime=SW_Ts
  Saturation : Saturate  UpperLimit=1  LowerLimit=-1
  Second-Order Filter : eeGeneralControl/Second-Order Filter  FilterType=Low-pass  fn=6000  Zeta=0.707  Ts=0  A0=0  Ph0=0  f0=0  b0=0
      settings: LibrarySourceBlock=ee_sl_lib/General Control/Second-Order Filter
  U_cmd : Outport
  wires:
  Gain4/1 -> Add3/1
  Memory/1 -> Second-Order Filter/1
  Second-Order Filter/1 -> Add2/2
  Saturation/1 -> U_cmd/1
  Add2/1 -> Ictrl_anti_windup/1(err), Gain4/1
  Add3/1 -> Saturation/1
  ref/1 -> Add2/1
  fbk/1 -> Rate Transition/1
  Rate Transition/1 -> Memory/1
  Ictrl_anti_windup/1(Int_out) -> Add3/2

== system Ten_phase_nine_leg_relocated_L3_L7/PI_ctrl8 ==
  ref : Inport
  fbk : Inport  Port=2
  Add2 : Sum  Inputs=+-
  Add3 : Sum
  Gain4 : Gain  Gain=K_p
  Ictrl_anti_windup : Subsystem
  Memory : Memory
  Rate Transition : RateTransition  OutPortSampleTime=SW_Ts
  Saturation : Saturate  UpperLimit=1  LowerLimit=-1
  Second-Order Filter : eeGeneralControl/Second-Order Filter  FilterType=Low-pass  fn=6000  Zeta=0.707  Ts=0  A0=0  Ph0=0  f0=0  b0=0
      settings: LibrarySourceBlock=ee_sl_lib/General Control/Second-Order Filter
  U_cmd : Outport
  wires:
  Gain4/1 -> Add3/1
  Memory/1 -> Second-Order Filter/1
  Second-Order Filter/1 -> Add2/2
  Saturation/1 -> U_cmd/1
  Add2/1 -> Ictrl_anti_windup/1(err), Gain4/1
  Add3/1 -> Saturation/1
  ref/1 -> Add2/1
  fbk/1 -> Rate Transition/1
  Rate Transition/1 -> Memory/1
  Ictrl_anti_windup/1(Int_out) -> Add3/2

== system Ten_phase_nine_leg_relocated_L3_L7/PI_ctrl9 ==
  ref : Inport
  fbk : Inport  Port=2
  Add2 : Sum  Inputs=+-
  Add3 : Sum
  Gain4 : Gain  Gain=K_p
  Ictrl_anti_windup : Subsystem
  Memory : Memory
  Rate Transition : RateTransition  OutPortSampleTime=SW_Ts
  Saturation : Saturate  UpperLimit=1  LowerLimit=-1
  Second-Order Filter : eeGeneralControl/Second-Order Filter  FilterType=Low-pass  fn=6000  Zeta=0.707  Ts=0  A0=0  Ph0=0  f0=0  b0=0
      settings: LibrarySourceBlock=ee_sl_lib/General Control/Second-Order Filter
  U_cmd : Outport
  wires:
  Gain4/1 -> Add3/1
  Memory/1 -> Second-Order Filter/1
  Second-Order Filter/1 -> Add2/2
  Saturation/1 -> U_cmd/1
  Add2/1 -> Ictrl_anti_windup/1(err), Gain4/1
  Add3/1 -> Saturation/1
  ref/1 -> Add2/1
  fbk/1 -> Rate Transition/1
  Rate Transition/1 -> Memory/1
  Ictrl_anti_windup/1(Int_out) -> Add3/2

== system Ten_phase_nine_leg_relocated_L3_L7/PWM_gen ==
  U : Inport
  Gain : Gain  Gain=15  OutDataTypeStr=double
  Gain1 : Gain  Gain=15  OutDataTypeStr=double
  NOT : Logic  Operator=NOT  IconShape=distinctive  AllPortsSameDT=off  OutDataTypeStr=boolean
  On-Off Delay : eeGeneralControl/On-Off Delay  LabelModeActiveChoice=Continuous  Td_on=1e-6  Td_off=0  IC=0  Ts=0
      settings: LibrarySourceBlock=ee_sl_lib/General Control/On-Off Delay
  On-Off Delay1 : eeGeneralControl/On-Off Delay  LabelModeActiveChoice=Continuous  Td_on=1e-6  Td_off=0  IC=0  Ts=0
      settings: LibrarySourceBlock=ee_sl_lib/General Control/On-Off Delay
  Relational Operator2 : RelationalOperator  OutDataTypeStr=boolean  RndMeth=Simplest  InputSameDT=off
  Repeating Sequence : simulink/Sources/Repeating Sequence  rep_seq_t=[0 half_SW_Ts SW_Ts]  rep_seq_y=[0 1 0]
  PWMH : Outport
  PWML : Outport  Port=2
  wires:
  Repeating Sequence/1 -> Relational Operator2/2
  U/1 -> Relational Operator2/1
  Relational Operator2/1 -> NOT/1, On-Off Delay1/1
  NOT/1 -> On-Off Delay/1
  On-Off Delay1/1 -> Gain/1
  Gain/1 -> PWMH/1
  On-Off Delay/1 -> Gain1/1
  Gain1/1 -> PWML/1

== system Ten_phase_nine_leg_relocated_L3_L7/PWM_gen1 ==
  U : Inport
  Gain : Gain  Gain=15  OutDataTypeStr=double
  Gain1 : Gain  Gain=15  OutDataTypeStr=double
  NOT : Logic  Operator=NOT  IconShape=distinctive  AllPortsSameDT=off  OutDataTypeStr=boolean
  On-Off Delay : eeGeneralControl/On-Off Delay  LabelModeActiveChoice=Continuous  Td_on=1e-6  Td_off=0  IC=0  Ts=0
      settings: LibrarySourceBlock=ee_sl_lib/General Control/On-Off Delay
  On-Off Delay1 : eeGeneralControl/On-Off Delay  LabelModeActiveChoice=Continuous  Td_on=1e-6  Td_off=0  IC=0  Ts=0
      settings: LibrarySourceBlock=ee_sl_lib/General Control/On-Off Delay
  Relational Operator2 : RelationalOperator  OutDataTypeStr=boolean  RndMeth=Simplest  InputSameDT=off
  Repeating Sequence : simulink/Sources/Repeating Sequence  rep_seq_t=[0 half_SW_Ts SW_Ts]  rep_seq_y=[0 1 0]
  PWMH : Outport
  PWML : Outport  Port=2
  wires:
  Repeating Sequence/1 -> Relational Operator2/2
  U/1 -> Relational Operator2/1
  Relational Operator2/1 -> NOT/1, On-Off Delay1/1
  NOT/1 -> On-Off Delay/1
  On-Off Delay1/1 -> Gain/1
  Gain/1 -> PWMH/1
  On-Off Delay/1 -> Gain1/1
  Gain1/1 -> PWML/1

== system Ten_phase_nine_leg_relocated_L3_L7/PWM_gen2 ==
  U : Inport
  Gain : Gain  Gain=15  OutDataTypeStr=double
  Gain1 : Gain  Gain=15  OutDataTypeStr=double
  NOT : Logic  Operator=NOT  IconShape=distinctive  AllPortsSameDT=off  OutDataTypeStr=boolean
  On-Off Delay : eeGeneralControl/On-Off Delay  LabelModeActiveChoice=Continuous  Td_on=1e-6  Td_off=0  IC=0  Ts=0
      settings: LibrarySourceBlock=ee_sl_lib/General Control/On-Off Delay
  On-Off Delay1 : eeGeneralControl/On-Off Delay  LabelModeActiveChoice=Continuous  Td_on=1e-6  Td_off=0  IC=0  Ts=0
      settings: LibrarySourceBlock=ee_sl_lib/General Control/On-Off Delay
  Relational Operator2 : RelationalOperator  OutDataTypeStr=boolean  RndMeth=Simplest  InputSameDT=off
  Repeating Sequence : simulink/Sources/Repeating Sequence  rep_seq_t=[0 half_SW_Ts SW_Ts]  rep_seq_y=[0 1 0]
  PWMH : Outport
  PWML : Outport  Port=2
  wires:
  Repeating Sequence/1 -> Relational Operator2/2
  U/1 -> Relational Operator2/1
  Relational Operator2/1 -> NOT/1, On-Off Delay1/1
  NOT/1 -> On-Off Delay/1
  On-Off Delay1/1 -> Gain/1
  Gain/1 -> PWMH/1
  On-Off Delay/1 -> Gain1/1
  Gain1/1 -> PWML/1

== system Ten_phase_nine_leg_relocated_L3_L7/PWM_gen3 ==
  U : Inport
  Gain : Gain  Gain=15  OutDataTypeStr=double
  Gain1 : Gain  Gain=15  OutDataTypeStr=double
  NOT : Logic  Operator=NOT  IconShape=distinctive  AllPortsSameDT=off  OutDataTypeStr=boolean
  On-Off Delay : eeGeneralControl/On-Off Delay  LabelModeActiveChoice=Continuous  Td_on=1e-6  Td_off=0  IC=0  Ts=0
      settings: LibrarySourceBlock=ee_sl_lib/General Control/On-Off Delay
  On-Off Delay1 : eeGeneralControl/On-Off Delay  LabelModeActiveChoice=Continuous  Td_on=1e-6  Td_off=0  IC=0  Ts=0
      settings: LibrarySourceBlock=ee_sl_lib/General Control/On-Off Delay
  Relational Operator2 : RelationalOperator  OutDataTypeStr=boolean  RndMeth=Simplest  InputSameDT=off
  Repeating Sequence : simulink/Sources/Repeating Sequence  rep_seq_t=[0 half_SW_Ts SW_Ts]  rep_seq_y=[0 1 0]
  PWMH : Outport
  PWML : Outport  Port=2
  wires:
  Repeating Sequence/1 -> Relational Operator2/2
  U/1 -> Relational Operator2/1
  Relational Operator2/1 -> NOT/1, On-Off Delay1/1
  NOT/1 -> On-Off Delay/1
  On-Off Delay1/1 -> Gain/1
  Gain/1 -> PWMH/1
  On-Off Delay/1 -> Gain1/1
  Gain1/1 -> PWML/1

== system Ten_phase_nine_leg_relocated_L3_L7/PWM_gen4 ==
  U : Inport
  Gain : Gain  Gain=15  OutDataTypeStr=double
  Gain1 : Gain  Gain=15  OutDataTypeStr=double
  NOT : Logic  Operator=NOT  IconShape=distinctive  AllPortsSameDT=off  OutDataTypeStr=boolean
  On-Off Delay : eeGeneralControl/On-Off Delay  LabelModeActiveChoice=Continuous  Td_on=1e-6  Td_off=0  IC=0  Ts=0
      settings: LibrarySourceBlock=ee_sl_lib/General Control/On-Off Delay
  On-Off Delay1 : eeGeneralControl/On-Off Delay  LabelModeActiveChoice=Continuous  Td_on=1e-6  Td_off=0  IC=0  Ts=0
      settings: LibrarySourceBlock=ee_sl_lib/General Control/On-Off Delay
  Relational Operator2 : RelationalOperator  OutDataTypeStr=boolean  RndMeth=Simplest  InputSameDT=off
  Repeating Sequence : simulink/Sources/Repeating Sequence  rep_seq_t=[0 half_SW_Ts SW_Ts]  rep_seq_y=[0 1 0]
  PWMH : Outport
  PWML : Outport  Port=2
  wires:
  Repeating Sequence/1 -> Relational Operator2/2
  U/1 -> Relational Operator2/1
  Relational Operator2/1 -> NOT/1, On-Off Delay1/1
  NOT/1 -> On-Off Delay/1
  On-Off Delay1/1 -> Gain/1
  Gain/1 -> PWMH/1
  On-Off Delay/1 -> Gain1/1
  Gain1/1 -> PWML/1
